simulink model "lab1_square_unreal"  (R2025b)
settings: Solver=ode4  StartTime=0.0  StopTime=13  FixedStep=0.01  RelTol=1e-3
model workspace (MAT data in the model file):
  SIDE = 2
  SPEED = 1
  TRACK = 0.3
  TURN_RATE = 1.57079632679
  WHEEL_ERROR = 0
  WHEEL_RADIUS = 0.05
libraries: sim3dlib x3, robotmobilelib x1
settings Model: Creator=xion  LastModifiedBy=xion

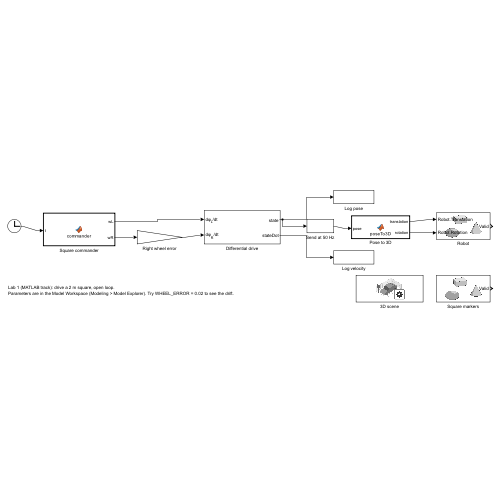
[thumbnail: Simulink's stored preview of the top-level diagram]
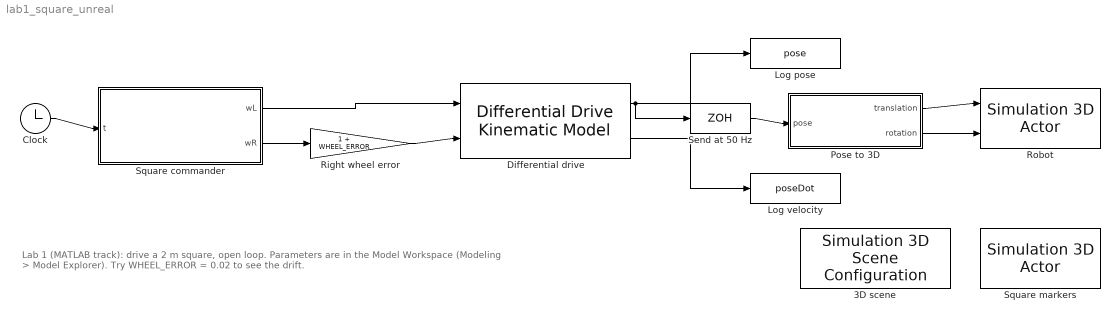
== system lab1_square_unreal ==
  note: Lab 1 (MATLAB track): drive a 2 m square, open loop.
      | Parameters are in the Model Workspace (Modeling > Model Explorer). Try WHEEL_ERROR = 0.02 to see the drift.
  3D scene : sim3dlib/Simulation 3D Scene Configuration  Priority=0  ProjectFormat=Default Scenes  SceneDesc=Open surface  ProjectName=D:\ProgramFiles\MATLAB\R2025b\toolbox\shared\sim3d_projects\automotive_project_windows\UE\WindowsNoEditor\VehicleSimulation.exe  ScenePath=/Game/Maps/HwStrght  EnableOpenDRIVE=off  vehTagList={'Custom';'Scene Origin'}  vehTag=Scene Origin  AttachedCameraRelativeTranslation=[0 0 0]  FreeCameraDefaultInitialTranslation=[-2.5, -1, 4.5]  AttachedCameraRelativeRotation=[0 0 0]  FreeCameraDefaultInitialRotation=[0, -50, 0]  ViewpointName=Custom  FreeCameraInitialTranslation=[-2.5, -1, 4.5]  ViewpointTranslation=[0 0 0]  FreeCameraInitialRotation=[0, -50, 0]  ViewpointRotation=[0 0 0]  OpVisEn=off  Ts=0.02  EnableWindow=on  EnableRemoteAccess=off  EnableWeather=off  SunAzimuth=90  SunAltitude=40.0  EnableGeospatialSun=off  Latitude=0  Longitude=0  Date=2023-01-01  Time=10:30:00  GeoTimeZone=-5.0  SunDaylightSaving=off  wind=1  clouds=10  EnableVolumetricClouds=off  CloudCoverage=0  CloudAltitude=6  fog=0  rain=0  RaindropsEffect=off  SnowDensity=0  EnableGeospatial=off  TilesetSource=Earth terrain  UseTrueOrigin=off  OriginHeight=200  OriginLatitude=40.744652  OriginLongitude=-73.988864  MapStyle=Aerial  AdditionalAssetIDs=[]  UseAdvancedSunSky=off  SolarTime=11  TimeZone=-5  Day=21  Month=9  Year=2022  UseDaylightSavingTime=on  DSTStartDay=10  DSTStartMonth=3  DSTEndDay=3  DSTEndMonth=11  DSTSwitchHour=2  sensorTag=MainCamera1  sensorId=1  sensorName=MainCamera1  mountLoc=Origin  offsetFlag=off  tmountOffset=[0, 0, 0]  rmountOffset=[0, 0, 0]  HorizontalResolution=1280  VerticalResolution=720  HorizontalFOV=60  mountPoint=[0 0 0]  mountOrientation=[0 0 0]  aMode=aMode  ID=1  GeoTrigger=Inactive  ViewNameList={'Custom'}  ViewTranslationList={'[-2.5 -1 4.5]'}  ViewRotationList={'[0 -50 0]'}
  Clock : Clock
  Differential drive : robotmobilelib/Differential Drive Kinematic Model  VehicleInputs=Wheel Speeds  WheelRadius=WHEEL_RADIUS  WheelSpeedRange=[-inf inf]  TrackWidth=TRACK  InitialState=[0; 0; 0]  SimulateUsing=Interpreted execution
  Log pose : ToWorkspace  VariableName=pose  SampleTime=-1
  Log velocity : ToWorkspace  VariableName=poseDot  SampleTime=-1
  Pose to 3D : MATLAB Function  TreatAsAtomicUnit=on
  Right wheel error : Gain  Gain=1 + WHEEL_ERROR
  Robot : sim3dlib/Simulation 3D Actor  Priority=1  ActorName=Robot  ParentName=Scene Origin  Operation=Create at setup  InitScriptText=|  SampleTime=0.02  Translation=[0 0 0]  Rotation=[0 0 0]  Scale=[1 1 1]  InputsText=Robot.Translation Robot.Rotation  aMode=aMode  ActorTag=Robot  ActorType=Sim3dActor  ID=C
      | % The robot: a cylinder body, a dome and a red nose that shows its heading
      | createShape(Actor, 'cylinder', [0.4 0.4 0.5]);
      | Actor.Color = [0.92 0.92 0.95];
      | dome = sim3d.Actor(ActorName='Dome');
      | createShape(dome, 'sphere', [0.4 0.4 0.4]);
      | dome.Color = [0.35 0.5 0.85];
      | dome.Translation = [0 0 0.25];
      | add(World, dome, Actor);
      | nose = sim3d.Actor(ActorName='Nose');
      | createShape(nose, 'box', [0.12 0.12 0.12]);
      | nose.Color = [0.85 0.1 0.1];
      | nose.Translation = [0.2 0 0.3];
      | add(World, nose, Actor);
  Send at 50 Hz : ZeroOrderHold  SampleTime=0.02
  Square commander : MATLAB Function  TreatAsAtomicUnit=on
  Square markers : sim3dlib/Simulation 3D Actor  Priority=1  ActorName=Markers  ParentName=Scene Origin  Operation=Create at setup  InitScriptText=|  SampleTime=0.02  Translation=[0 0 0]  Rotation=[0 0 0]  Scale=[1 1 1]  aMode=aMode  ActorTag=Markers  ActorType=Sim3dActor  ID=C
      | % A tiny base at the origin; the lines and posts are its children
      | createShape(Actor, 'box', [0.01 0.01 0.01]);
      | corners = [0 0; 2 0; 2 -2; 0 -2];   % the square in Unreal's frame (y flipped)
      | for k = 1:4
      |     post = sim3d.Actor(ActorName=sprintf('Post%d', k));
      |     createShape(post, 'cylinder', [0.08 0.08 0.4]);
      |     post.Color = [0.95 0.55 0.1];
      |     post.Translation = [corners(k, :), 0.2];
      |     add(World, post, Actor);
      |     a = corners(k, :);
      |     b = corners(mod(k, 4) + 1, :);
      |     edge = sim3d.Actor(ActorName=sprintf('Edge%d', k));
      |     createShape(edge, 'box', [norm(b - a) + 0.05, 0.05, 0.01]);
      |     edge.Color = [1 1 1];
      |     edge.Translation = [(a + b) / 2, 0.005];
      |     edge.Rotation = [0, 0, atan2(b(2) - a(2), b(1) - a(1))];
      |     add(World, edge, Actor);
      | end
  wires:
  Clock/1 -> Square commander/1(t)
  Square commander/1(wL) -> Differential drive/1
  Square commander/2(wR) -> Right wheel error/1
  Right wheel error/1 -> Differential drive/2
  Differential drive/1 -> Log pose/1, Send at 50 Hz/1
  Differential drive/2 -> Log velocity/1
  Send at 50 Hz/1 -> Pose to 3D/1(pose)
  Pose to 3D/1(translation) -> Robot/1
  Pose to 3D/2(rotation) -> Robot/2

== matlab function lab1_square_unreal/Pose to 3D ==
  data: pose input; translation output; rotation output
function [translation, rotation] = poseTo3D(pose)
% pose = [x; y; theta] from the drive block -> the actor's position and rotation.
% Unreal's world is left-handed (y points right), so y and the heading change sign:
% otherwise every left turn would look like a right turn on the screen.
translation = [pose(1), -pose(2), 0.25];  % lift the body so it stands on the floor, m
rotation = [0, 0, -pose(3)];              % roll, pitch, yaw, rad

== matlab function lab1_square_unreal/Square commander ==
  data: t input; wL output; wR output; SIDE parameter; SPEED parameter; TURN_RATE parameter; WHEEL_RADIUS parameter; TRACK parameter
function [wL, wR] = commander(t, SIDE, SPEED, TURN_RATE, WHEEL_RADIUS, TRACK)
% Open-loop square, as in the Python lab: drive SIDE metres, turn 90 degrees left,
% four times, then stop. No sensor is used: the robot does not know where it is.
tSide = SIDE / SPEED;            % time to drive one side, s
tTurn = (pi/2) / TURN_RATE;      % time to turn 90 degrees, s
period = tSide + tTurn;
if t >= 4 * period
    v = 0; w = 0;                % finished: stop
elseif mod(t, period) < tSide
    v = SPEED; w = 0;            % drive forward
else
    v = 0; w = TURN_RATE;        % turn left on the spot
end
% Inverse kinematics of a differential drive: body speeds -> wheel speeds (rad/s)
wL = (v - w * TRACK / 2) / WHEEL_RADIUS;
wR = (v + w * TRACK / 2) / WHEEL_RADIUS;
